simulink model "Terasic_Hinf_2PWM"  (R2024b)
settings: Solver=VariableStepAuto  StartTime=0.0  StopTime=40  RelTol=1e-3  AbsTol=1e-3  EnableMultiTasking=on
model workspace (MAT data in the model file):
  A = [0 0 0 0 0 0 0 0 0 46.1581109565 55.047620673 0 ... (36 elements, 6x6)]
  A_d = [1 0 0 0 0 0 0.00231129246651 1.00275236665 0 0.462701764161 0.550598858215 0 ... (36 elements, 6x6)]
  Ak = [1.00039205 -0.000215147789448 -1.64001804099e-18 0.0780748009937 -0.0428745691318 -3.25813654462e-16 1 0 0 0 0 0 ... (144 elements, 12x12)]
  B = [0  0; 0  0; 0  0; 27.6621403954  27.6621403954; -15.1701338659  -15.1701338659; 16.6718431468  -16.6718431468]
  B_d = [0.00137160104409  0.00137160104409; -0.00075270229638  -0.00075270229638; 0.000826833699011  -0.000826833699011; 0.27314750548  0.27314750548; -0.14999822552  -0.14999822552; 0.164695013627  -0.164695013627]
  Bk = [0.00897508903654 0.000996461505483 1.10454949677e-17 0.0192045376467 0.00234293304406 5.68718242914e-17 0.00885401920589 0.000938057760568 1.07064637708e-17 0.00495786380359 0.00937391189217 4.84377922718e-17 ... (72 elements, 12x6)]
  C = [1 0 0 0 0 0 0 1 0 0 0 0 ... (36 elements, 6x6)]
  C_d = [1 0 0 0 0 0 0 1 0 0 0 0 ... (36 elements, 6x6)]
  Ck = [0.153095590413 0.153095590413 11.9137808131 11.9137808131 -1.20372110104 1.20372110104 0.27169183822 0.27169183822 1.38991961251 1.38991961251 -0.273777490273 0.273777490273 ... (24 elements, 2x12)]
  D = [0  0; 0  0; 0  0; 0  0; 0  0; 0  0]
  D_mech = [0.0252  -0.0252  0; -0.0252  0.0252  0; 0  0  0.166281609375]
  Dk = [0.0269073209626  13.1663391007  -0.0805689409227  -0.0333464874403  1.30114752723  -0.0564338780901; 0.0269073209626  13.1663391007  0.0805689409227  -0.0333464874403  1.30114752723  0.0564338780901]
  G = [1  1; -1  -1; 2.56875  -2.56875]
  I_stall = 1
  Ip = 0.00145
  Iz = 0.00097
  Jm = 0.005
  Jw = 2.5088e-05
  K_dlqr = [-0.853251287852  -36.6769630694  1.12869840177  -1.09321384812  -4.23786339844  1.08671927262; -0.853251287852  -36.6769630694  -1.12869840177  -1.09321384812  -4.23786339844  -1.08671927262]
  K_mech = [0  0  0; 0  -0.2584205136  0; 0  0  0]
  M = [0.010920576  -0.00915703808  0; -0.00915703808  0.0123727798768  0; 0  0  0.067948021105]
  N = [0  0; 0  0; 0  0; 0  0; 0  0; 0  0]
  P_dlqr = [5005.96418436 19209.6778099 -1.2921851815e-11 1093.04425821 2096.5541522 1.75770983653e-12 19209.6778099 419963.763285 -8.32375733119e-10 21774.9396257 43954.8588772 1.78984289418e-11 ... (36 elements, 6x6)]
  Q = [40.12 0 0 0 0 0 0 40.18 0 0 0 0 ... (36 elements, 6x6)]
  R = [10  0; 0  10]
  R_int = 12
  V_nom = 12
  b = 0.1644
  c = 0.0126
  chassis_I_diag = [0.000895 0.00145 0.00097]
  chassis_I_prod = [9e-06 -4e-06 2.1e-05]
  chassis_com = [0.0003 0.00053 0.03503]
  chassis_mass = 0.752
  d = 2.56875
  dt = 0.01
  g = 9.81
  gear = 30
  half_track_over_radius = 2.56875
  hinf_x0 = [0; 0; 0; 0; 0; 0; 0; 0; 0; 0; 0; 0]
  joint_damping = 0.0126
  joint_friction = 0.01
  k_t = 0.0147
  l = 0.03503
  m = 0.752
  max_pwm = 0.15
  motor_max_torque = 0.441
  mu_kinematic = 0.5
  mu_static = 0.6
  mw = 0.049
  poles_dlqr = [0.990060810875+0i; 0.99004694653+0i; 0.921689587164+0.0192903791613i; 0.921689587164-0.0192903791613i; 0.625943331335+0i; 0.420899120063+0i]
  r = 0.032
  rotor_inertia = 0.005
  rotor_inertia_per_wheel = 0.005
  sigma_pitch_encoder = -1
  sys_dlqr : object (value not decoded)
  torque_per_pwm = 0.441
  wheel_inertia = 2.5088e-05
  wheel_mass = 0.049
  wheel_offset_x = 0.082
  wheel_radius = 0.032
  wheel_thickness = 0.028
  wheel_track = 0.1644
undefined symbols (not defined in the file or in its folder): X, Y, Z
libraries: sm_lib x29, nesl_utility x18, simulink x2
(part 2 of 2)

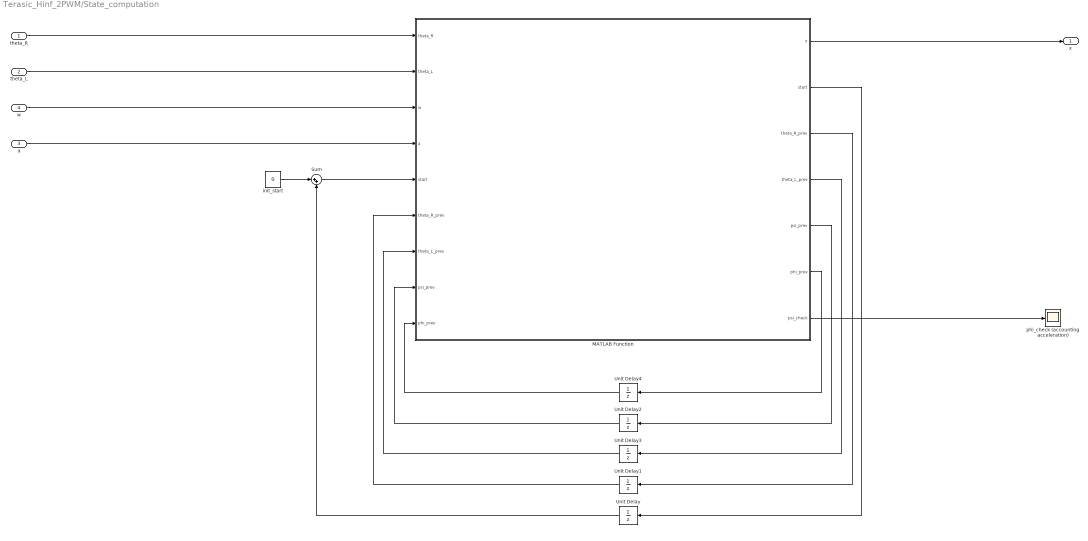
== system Terasic_Hinf_2PWM/State_computation ==
  theta_R : Inport
  theta_L : Inport  Port=2
  a : Inport  Port=3
  w : Inport  Port=4
  MATLAB Function : MATLAB Function  TreatAsAtomicUnit=on
  Sum : Sum  Inputs=|++
  Unit Delay{,1..4} (5 alike) : UnitDelay  SampleTime=dt  HasFrameUpgradeWarning=on
  init_start : Constant  Value=0
  phi_check (accounting acceleration) : Scope
  x : Outport
  wires:
  theta_L/1 -> MATLAB Function/2(theta_L)
  MATLAB Function/3(theta_R_prev) -> Unit Delay1/1
  Unit Delay1/1 -> MATLAB Function/6("theta_R_prev ")
  theta_R/1 -> MATLAB Function/1(theta_R)
  Unit Delay/1 -> Sum/2
  MATLAB Function/4(theta_L_prev) -> Unit Delay3/1
  Unit Delay3/1 -> MATLAB Function/7("theta_L_prev ")
  MATLAB Function/2(start) -> Unit Delay/1
  init_start/1 -> Sum/1
  Sum/1 -> MATLAB Function/5("start ")
  MATLAB Function/1(x) -> x/1
  w/1 -> MATLAB Function/3(w)
  a/1 -> MATLAB Function/4(a)
  MATLAB Function/5(psi_prev) -> Unit Delay2/1
  Unit Delay2/1 -> MATLAB Function/8("psi_prev ")
  MATLAB Function/6(phi_prev) -> Unit Delay4/1
  Unit Delay4/1 -> MATLAB Function/9("phi_prev ")
  MATLAB Function/7(psi_check) -> phi_check (accounting acceleration)/1

== matlab function Terasic_Hinf_2PWM/State_computation/MATLAB Function ==
  data: theta_R input; x output; theta_L input; w input; a input; start input; theta_R_prev input; theta_L_prev input; wheel_radius parameter; wheel_track parameter; dt parameter; psi_prev input; start output; theta_R_prev output; theta_L_prev output; psi_prev output; phi_prev input; phi_prev output; psi_check output
function [x, start, theta_R_prev, theta_L_prev, psi_prev, phi_prev, psi_check] = ...
    state_estimator(theta_R, theta_L, w, a, ...
                    start, theta_R_prev, theta_L_prev, wheel_radius, wheel_track, dt, psi_prev, phi_prev)
psi_check = 0;
% STATE_ESTIMATOR
% Vettore di stato:
%   x = [theta; psi; phi; theta_dot; psi_dot; phi_dot]
%
% theta_R, theta_L : angoli encoder delle ruote [rad]
% psi        : posizione del giunto di pitch [rad]
% psi_dot   : velocità del giunto di pitch [rad/s]
% start            : flag di inizializzazione
% theta_R_prev,
% theta_L_prev     : angoli delle ruote al campione precedente [rad]
% wheel_radius     : raggio ruota [m]
% wheel_track      : distanza tra le ruote [m]
% dt               : intervallo di campionamento [s]


    % Protezione da parametri non validi
    if dt <= 0 || wheel_track == 0
        x = zeros(6,1);
        return;
    end

    % Inizializza le memorie degli encoder senza generare un picco
    % artificiale di velocità al primo campione.
    if start == 0
        theta_R_prev = theta_R;
        theta_L_prev = theta_L;
        psi_prev = 0;
        phi_prev = 0;
        start = 1;
    end

    % Velocità angolari delle ruote da differenza discreta
    theta_R_dot = (theta_R - theta_R_prev) / dt;
    theta_L_dot = (theta_L - theta_L_prev) / dt;

    % Aggiorna le memorie per il campione successivo
    theta_R_prev = theta_R;
    theta_L_prev = theta_L;

    % Pitch_dot ottenuto dall'IMU
    psi_dot = -w(1);  % it's the pitch_dot detected

    % Pitch computation
    %%% IT NEEDS KALMAN FILTER FOR THE NOISE, BUT IT'S MORE ACCURATE
    %%% ACCOUNTING THE ACCELERATION
    psi_acc = -atan2(a(3), a(1));

    alpha = 0.99;
    psi_comp = alpha * (psi_prev + psi_dot * dt) ...
        + (1 - alpha) * psi_acc;
    psi_check = psi_comp;
    
    psi = psi_prev + psi_dot * dt;

    psi_prev = psi;


    % Rotazione media delle ruote
    theta_enc_mean = (theta_R + theta_L) / 2;
    theta_enc_dot  = (theta_R_dot + theta_L_dot) / 2;

    theta     = theta_enc_mean + psi;
    theta_dot = theta_enc_dot  + psi_dot;

    % Yaw ricavato dalla IMU
    % phi = (wheel_radius / wheel_track) * (theta_R - theta_L);
    % phi_dot = (wheel_radius / wheel_track) * ...
    %           (theta_R_dot - theta_L_dot);
    phi_dot = -w(3);
    phi = phi_prev + phi_dot * dt;
    phi_prev = phi;

    % Ordine richiesto dal controllore
    x = [theta;
         psi;
         phi;
         theta_dot;
         psi_dot;
         phi_dot];
end
